simulink model "inverted_pendulum"  (R2023b)
settings: Solver=VariableStepAuto  StartTime=0.0  StopTime=100  MaxStep=0.001  RelTol=1e-3
libraries: simulink_extras x1, slpidlib x1
settings Model: Creator=B03-402  LastModifiedBy=HP

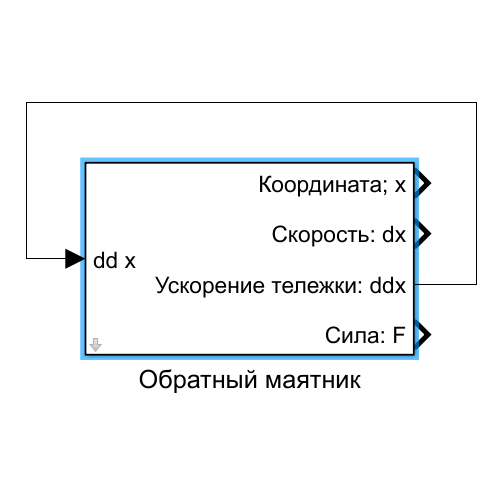
[thumbnail: Simulink's stored preview of the top-level diagram]
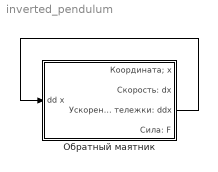
== system inverted_pendulum ==
  Обратный маятник : Subsystem  mask{L=0.8, m=0.3, mbig=20, b=0}
      mask prompts: L "Длина подвеса, м"; m "Масса подвеса, кг"; mbig "Масса тележки, кг"; b "Коэффициент диссипативных сил"
  wires:
  Обратный маятник/3(Ускорение тележки: ddx) -> Обратный маятник/1(dd x)

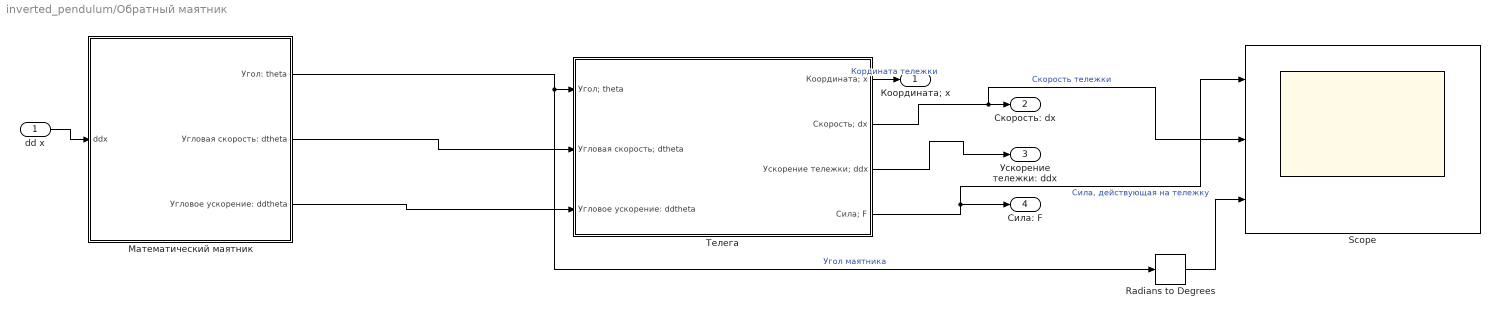
== system inverted_pendulum/Обратный маятник ==
  dd x : Inport
  Radians to Degrees : simulink_extras/Transformations/Radians to Degrees
  Scope : Scope  NumInputPorts=3
  Математический маятник : Subsystem
  Телега : Subsystem
  Координата; x : Outport
  Скорость: dx : Outport  Port=2
  Ускорение тележки: ddx : Outport  Port=3
  Сила: F : Outport  Port=4
  wires:
  Телега/1(Координата; x) -> Координата; x/1  "Кордината тележки"
  Математический маятник/2(Угловая скорость: dtheta) -> Телега/2(Угловая скорость; dtheta)
  Математический маятник/3(Угловое ускорение: ddtheta) -> Телега/3(Угловое ускорение: ddtheta)
  Телега/3(Ускорение тележки; ddx) -> Ускорение тележки: ddx/1
  Математический маятник/1(Угол: theta) -> Radians to Degrees/1, Телега/1(Угол; theta)  "Угол маятника"
  Телега/4(Сила; F) -> Scope/1, Сила: F/1  "Сила, действующая на тележку"
  Телега/2(Скорость; dx) -> Scope/2, Скорость: dx/1  "Скорость тележки"
  dd x/1 -> Математический маятник/1(ddx)
  Radians to Degrees/1 -> Scope/3

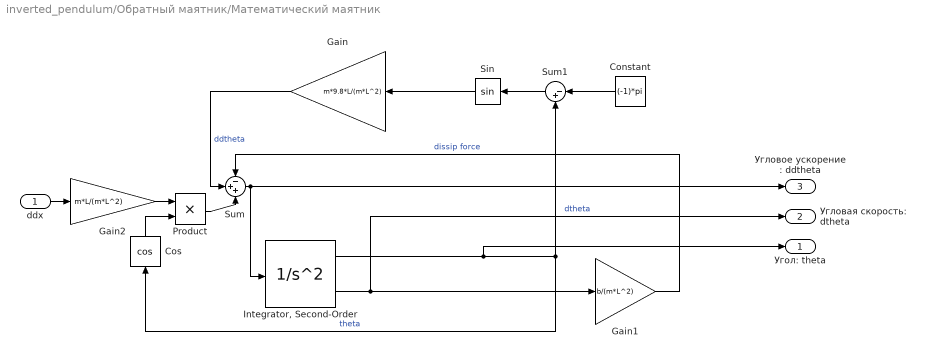
== system inverted_pendulum/Обратный маятник/Математический маятник ==
  ddx : Inport
  Constant : Constant  Value=(-1)*pi
  Cos : Trigonometry  Operator=cos
  Gain : Gain  Gain=m*9.8*L/(m*L^2)
  Gain1 : Gain  Gain=b/(m*L^2)
  Gain2 : Gain  Gain=m*L/(m*L^2)
  "Integrator, Second-Order" : SecondOrderIntegrator  ICX=deg2rad(20)
  Product : Product
  Sin : Trigonometry
  Sum : Sum  Inputs=-++
  Sum1 : Sum  Inputs=|-+
  Угол: theta : Outport
  Угловая скорость: dtheta : Outport  Port=2
  Угловое ускорение: ddtheta : Outport  Port=3
  wires:
  Gain1/1 -> Sum/1  "dissip force"
  "Integrator, Second-Order"/2 -> Gain1/1, Угловая скорость: dtheta/1  "dtheta"
  Sin/1 -> Gain/1
  Sum/1 -> "Integrator, Second-Order"/1, Угловое ускорение: ddtheta/1
  "Integrator, Second-Order"/1 -> Угол: theta/1, Sum1/2, Cos/1  "theta"
  Gain/1 -> Sum/2  "ddtheta"
  ddx/1 -> Gain2/1
  Gain2/1 -> Product/1
  Cos/1 -> Product/2
  Product/1 -> Sum/3
  Sum1/1 -> Sin/1
  Constant/1 -> Sum1/1

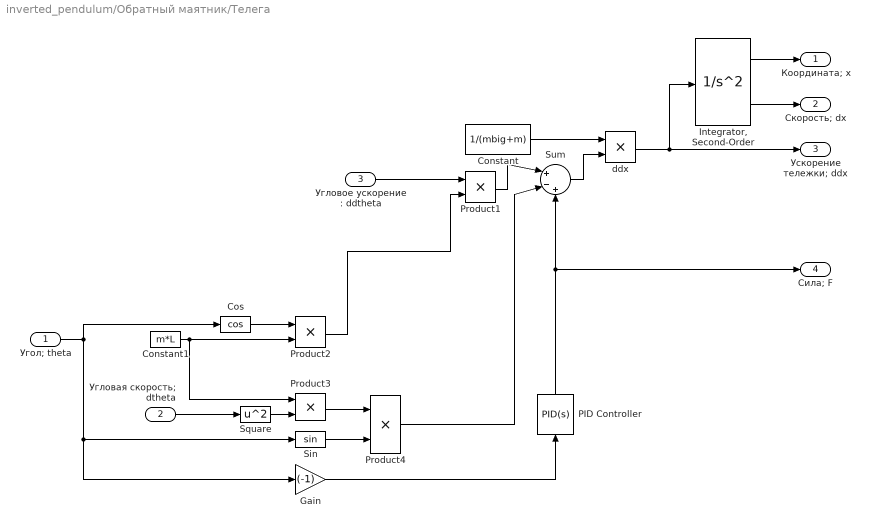
== system inverted_pendulum/Обратный маятник/Телега ==
  Угол; theta : Inport
  Угловая скорость; dtheta : Inport  Port=2
  Угловое ускорение: ddtheta : Inport  Port=3
  Constant : Constant  Value=1/(mbig+m)
  Constant1 : Constant  Value=m*L
  Cos : Trigonometry  Operator=cos
  Gain : Gain  Gain=(-1)
  "Integrator, Second-Order" : SecondOrderIntegrator
  PID Controller : slpidlib/PID Controller  Controller=PID  Form=Parallel  TimeDomain=Continuous-time  UseExternalTs=off  SampleTime=-1  IntegratorMethod=Forward Euler  FilterMethod=Forward Euler  ControllerParametersSource=internal  P=1  I=1  UseKiTs=off  D=23  N=100  UseFilter=on  TunerSelectOption=Transfer Function Based (PID Tuner App)  InitialConditionSource=internal  InitialConditionForIntegrator=0  InitialConditionForFilter=0  DifferentiatorICPrevScaledInput=0  ExternalReset=none  TrackingMode=off  Kt=1  LimitOutput=off  SatLimitsSource=internal  UpperSaturationLimit=inf  LowerSaturationLimit=-inf  LinearizeAsGain=on  AntiWindupMode=none  Kb=1  LimitIntegrator=off  UpperIntegratorSaturationLimit=inf  LowerIntegratorSaturationLimit=-inf  POutMin=[]  POutMax=[]  IOutMin=[]  IOutMax=[]  DOutMin=[]  DOutMax=[]  NOutMin=[]  NOutMax=[]  SumOutMin=[]  SumOutMax=[]  SaturationOutMin=[]  SaturationOutMax=[]  PParamMin=[]  PParamMax=[]  IParamMin=[]  IParamMax=[]  DParamMin=[]  DParamMax=[]  NParamMin=[]  NParamMax=[]  KbParamMin=[]  KbParamMax=[]  KtParamMin=[]  KtParamMax=[]  KbOutMin=[]  KbOutMax=[]  KtOutMin=[]  KtOutMax=[]  IntegratorOutMin=[]  IntegratorOutMax=[]  FilterOutMin=[]  FilterOutMax=[]  SumI1OutMin=[]  SumI1OutMax=[]  SumI2OutMin=[]  SumI2OutMax=[]  SumI3OutMin=[]  SumI3OutMax=[]  SumI4OutMin=[]  SumI4OutMax=[]  SumDOutMin=[]  SumDOutMax=[]  DifferentiatorOutMin=[]  DifferentiatorOutMax=[]  FilterDiffOutCoefMin=[]  FilterDiffOutCoefMax=[]  ReciprocalOutMin=[]  ReciprocalOutMax=[]  SumDenOutMin=[]  SumDenOutMax=[]  SumNumOutMin=[]  SumNumOutMax=[]  DivideOutMin=[]  DivideOutMax=[]  UdiffTsProdOutMin=[]  UdiffTsProdOutMax=[]  NTsProdOutMin=[]  NTsProdOutMax=[]  UintegralTsProdOutMin=[]  UintegralTsProdOutMax=[]  UngainTsProdOutMin=[]  UngainTsProdOutMax=[]  ClampingZeroOutDataTypeStr=Inherit: Inherit via back propagation  ClampingZeroOutMin=[]  ClampingZeroOutMax=[]  FilterDenConstantOutDataTypeStr=Inherit: Inherit via back propagation  FilterDenConstantOutMin=[]  FilterDenConstantOutMax=[]  PCopyOutDataTypeStr=Inherit: Inherit via back propagation  PCopyOutMin=[]  PCopyOutMax=[]  NCopyOutDataTypeStr=Inherit: Inherit via back propagation  NCopyOutMin=[]  NCopyOutMax=[]  IntegratorContinuousStateAttributes=''  IntegratorStateMustResolveToSignalObject=off  IntegratorRTWStateStorageClass=Auto  FilterContinuousStateAttributes=''  FilterStateMustResolveToSignalObject=off  FilterRTWStateStorageClass=Auto  ParallelPVariant=InternalParameters  IdealPVariant=Disabled  IVariant=InternalParameters  DVariant=InternalParameters  IntegratorVariant=Continuous  SatVariant=Disabled  AWVariant=Passthrough  PCopyVariant=Disabled  TRVariant=Disabled  FdbkBlocksVariant=Forward  IdealPFdbkVariant=Disabled  SatFdbkVariant=Disabled  DerivativeFilterVariant=ContFilter  NVariant=InternalParameters  NCopyVariant=Disabled  FilterICVariant=InternalICsFilter  IntegratorICVariant=InternalICs  ExternalResetVariant=Disabled  TRSumVariant=Passthrough  SumFdbkVariant=Disabled  SumVariant=Sum_PID  TsampFilterVariant=InternalTs  TsampNgainVariant=Passthrough  TsampIntegralVariant=Disabled_SignalSpec  ExternalSaturationOutDataTypeStr=Inherit: Same as second input
  Product{1..4} (4 alike) : Product
  Sin : Trigonometry
  Square : Math  Operator=square
  Sum : Sum  Inputs=|+-+
  ddx : Product
  Координата; x : Outport
  Скорость; dx : Outport  Port=2
  Ускорение тележки; ddx : Outport  Port=3
  Сила; F : Outport  Port=4
  wires:
  Constant/1 -> ddx/1
  Constant1/1 -> Product3/1, Product2/2
  Угловое ускорение: ddtheta/1 -> Product1/1
  Product2/1 -> Product1/2
  Угол; theta/1 -> Gain/1, Sin/1, Cos/1
  Cos/1 -> Product2/1
  Product1/1 -> Sum/1
  Угловая скорость; dtheta/1 -> Square/1
  Square/1 -> Product3/2
  Product3/1 -> Product4/1
  Sin/1 -> Product4/2
  Product4/1 -> Sum/2
  Sum/1 -> ddx/2
  ddx/1 -> "Integrator, Second-Order"/1, Ускорение тележки; ddx/1
  "Integrator, Second-Order"/1 -> Координата; x/1
  "Integrator, Second-Order"/2 -> Скорость; dx/1
  PID Controller/1 -> Sum/3, Сила; F/1
  Gain/1 -> PID Controller/1
